simulink model "talos_navigation"  (R2023a)
settings: Solver=FixedStepDiscrete  StartTime=0.0  StopTime=10.0  FixedStep=1/1000.0  RelTol=1e-3  EnableMultiTasking=on
undefined symbols (not defined in the file): accel, child_frame_id, child_frame_id_SL_Info, data, data_SL_Info, header, layout, transform, transforms, transforms_SL_Info
libraries: ros2lib x187, simulink x9, sharedTrackingLibrary x1
(part 1 of 3)
settings Model: Creator=ethan  LastModifiedBy=ethan
settings OptimizationCC: DefaultParameterBehavior=Inlined  EnhancedBackFolding=on  PassReuseOutputArgsAs=Individual arguments  ZeroExternalMemoryAtStartup=off  ZeroInternalMemoryAtStartup=off  OptimizeBlockOrder=speed  DifferentSizesBufferReuse=on  OptimizationCustomize=off  EfficientTunableParamExpr=on
settings DebuggingCC: ParameterTunabilityLossMsg=error
settings SFSimCC: MATLABDynamicMemAlloc=off
settings RTWCC: Description=Embedded Coder  SystemTargetFile=ert.tlc  TemplateMakefile=ert_default_tmf  CustomInitializer=talos_nav_start_wake_timer();  CustomTerminator=talos_nav_release_ros();
settings RTWCC: CustomSourceCode=|
  | #include <chrono>
  | #include <new>
  | 
  | template<class T>
  | static void talos_nav_release(T & entity)
  | {
  |   entity.~T();
  |   new (&entity) T();
  | }
  | 
  | static rclcpp::CallbackGroup::SharedPtr talos_nav_wake_group;
  | static rclcpp::TimerBase::SharedPtr talos_nav_wake_timer;
  | 
  | static void talos_nav_start_wake_timer()
  | {
  |   talos_nav_wake_group = SLROSNodePtr->create_callback_group(rclcpp::CallbackGroupType::Reentrant);
  |   talos_nav_wake_timer = SLROSNodePtr->create_wall_timer(
  |     std::chrono::milliseconds(10), []() {}, talos_nav_wake_group);
  | }
  | 
  | static void talos_nav_release_ros()
  | {
  |   talos_nav_wake_timer.reset();
  |   talos_nav_wake_group.reset();
  |   talos_nav_release(Pub_talos_navigation_776);
  |   talos_nav_release(Pub_talos_navigation_825);
  |   talos_nav_release(Pub_talos_navigation_838);
  |   talos_nav_release(Pub_talos_navigation_751);
  |   talos_nav_release(Pub_talos_navigation_804);
  |   talos_nav_release(Sub_talos_navigation_275);
  |   talos_nav_release(Sub_talos_navigation_273);
  |   talos_nav_release(Sub_talos_navigation_271);
  |   talos_nav_release(Sub_talos_navigation_269);
  |   talos_nav_release(Sub_talos_navigation_277);
  |   talos_nav_release(ParamGet_talos_navigation_254);
  |   talos_nav_release(ParamGet_talos_navigation_252);
  |   talos_nav_release(ParamGet_talos_navigation_253);
  |   talos_nav_release(ParamGet_talos_navigation_255);
  |   talos_nav_release(ParamGet_talos_navigation_168);
  |   talos_nav_release(ParamGet_talos_navigation_171);
  |   talos_nav_release(ParamGet_talos_navigation_172);
  |   talos_nav_release(ParamGet_talos_navigation_173);
  |   talos_nav_release(ParamGet_talos_navigation_175);
  |   talos_nav_release(ParamGet_talos_navigation_177);
  |   talos_nav_release(ParamGet_talos_navigation_176);
  |   talos_nav_release(ParamGet_talos_navigation_167);
  |   talos_nav_release(ParamGet_talos_navigation_179);
  |   talos_nav_release(ParamGet_talos_navigation_178);
  |   talos_nav_release(ParamGet_talos_navigation_221);
  |   talos_nav_release(ParamGet_talos_navigation_219);
  |   talos_nav_release(ParamGet_talos_navigation_220);
  |   talos_nav_release(ParamGet_talos_navigation_218);
  |   talos_nav_release(ParamGet_talos_navigation_165);
  |   talos_nav_release(ParamGet_talos_navigation_182);
  |   talos_nav_release(ParamGet_talos_navigation_183);
  |   talos_nav_release(ParamGet_talos_navigation_192);
  |   talos_nav_release(ParamGet_talos_navigation_193);
  |   talos_nav_release(ParamGet_talos_navigation_194);
  |   talos_nav_release(ParamGet_talos_navigation_195);
  |   talos_nav_release(ParamGet_talos_navigation_196);
  |   talos_nav_release(ParamGet_talos_navigation_197);
  |   talos_nav_release(ParamGet_talos_navigation_184);
  |   talos_nav_release(ParamGet_talos_navigation_185);
  |   talos_nav_release(ParamGet_talos_navigation_186);
  |   talos_nav_release(ParamGet_talos_navigation_187);
  |   talos_nav_release(ParamGet_talos_navigation_188);
  |   talos_nav_release(ParamGet_talos_navigation_189);
  |   talos_nav_release(ParamGet_talos_navigation_190);
  |   talos_nav_release(ParamGet_talos_navigation_191);
  |   talos_nav_release(ParamGet_talos_navigation_201);
  |   talos_nav_release(ParamGet_talos_navigation_202);
  |   talos_nav_release(ParamGet_talos_navigation_211);
  |   talos_nav_release(ParamGet_talos_navigation_212);
  |   talos_nav_release(ParamGet_talos_navigation_213);
  |   talos_nav_release(ParamGet_talos_navigation_214);
  |   talos_nav_release(ParamGet_talos_navigation_215);
  |   talos_nav_release(ParamGet_talos_navigation_216);
  |   talos_nav_release(ParamGet_talos_navigation_203);
  |   talos_nav_release(ParamGet_talos_navigation_204);
  |   talos_nav_release(ParamGet_talos_navigation_205);
  |   talos_nav_release(ParamGet_talos_navigation_206);
  |   talos_nav_release(ParamGet_talos_navigation_207);
  |   talos_nav_release(ParamGet_talos_navigation_208);
  |   talos_nav_release(ParamGet_talos_navigation_209);
  |   talos_nav_release(ParamGet_talos_navigation_210);
  |   talos_nav_release(ParamGet_talos_navigation_222);
  |   talos_nav_release(ParamGet_talos_navigation_166);
  |   talos_nav_release(ParamGet_talos_navigation_7);
  |   talos_nav_release(ParamGet_talos_navigation_14);
  |   talos_nav_release(ParamGet_talos_navigation_12);
  |   talos_nav_release(ParamGet_talos_navigation_10);
  |   talos_nav_release(ParamGet_talos_navigation_9);
  |   talos_nav_release(ParamGet_talos_navigation_5);
  |   talos_nav_release(ParamGet_talos_navigation_227);
  |   talos_nav_release(ParamGet_talos_navigation_240);
  |   talos_nav_release(ParamGet_talos_navigation_226);
  |   talos_nav_release(ParamGet_talos_navigation_241);
  |   talos_nav_release(ParamGet_talos_navigation_242);
  |   talos_nav_release(ParamGet_talos_navigation_229);
  |   talos_nav_release(ParamGet_talos_navigation_230);
  |   talos_nav_release(ParamGet_talos_navigation_235);
  |   talos_nav_release(ParamGet_talos_navigation_236);
  |   talos_nav_release(ParamGet_talos_navigation_237);
  |   talos_nav_release(ParamGet_talos_navigation_238);
  |   talos_nav_release(ParamGet_talos_navigation_244);
  |   talos_nav_release(ParamGet_talos_navigation_248);
  |   talos_nav_release(ParamGet_talos_navigation_247);
  |   talos_nav_release(ParamGet_talos_navigation_243);
  |   talos_nav_release(ParamGet_talos_navigation_245);
  |   talos_nav_release(ParamGet_talos_navigation_246);
  |   talos_nav_release(ParamGet_talos_navigation_232);
  |   talos_nav_release(ParamGet_talos_navigation_228);
  |   talos_nav_release(ParamGet_talos_navigation_231);
  |   talos_nav_release(ParamGet_talos_navigation_62);
  |   talos_nav_release(ParamGet_talos_navigation_64);
  |   talos_nav_release(ParamGet_talos_navigation_73);
  |   talos_nav_release(ParamGet_talos_navigation_74);
  |   talos_nav_release(ParamGet_talos_navigation_75);
  |   talos_nav_release(ParamGet_talos_navigation_76);
  |   talos_nav_release(ParamGet_talos_navigation_67);
  |   talos_nav_release(ParamGet_talos_navigation_68);
  |   talos_nav_release(ParamGet_talos_navigation_69);
  |   talos_nav_release(ParamGet_talos_navigation_48);
  |   talos_nav_release(ParamGet_talos_navigation_57);
  |   talos_nav_release(ParamGet_talos_navigation_58);
  |   talos_nav_release(ParamGet_talos_navigation_59);
  |   talos_nav_release(ParamGet_talos_navigation_60);
  |   talos_nav_release(ParamGet_talos_navigation_51);
  |   talos_nav_release(ParamGet_talos_navigation_52);
  |   talos_nav_release(ParamGet_talos_navigation_53);
  |   talos_nav_release(ParamGet_talos_navigation_34);
  |   talos_nav_release(ParamGet_talos_navigation_43);
  |   talos_nav_release(ParamGet_talos_navigation_44);
  |   talos_nav_release(ParamGet_talos_navigation_45);
  |   talos_nav_release(ParamGet_talos_navigation_46);
  |   talos_nav_release(ParamGet_talos_navigation_37);
  |   talos_nav_release(ParamGet_talos_navigation_38);
  |   talos_nav_release(ParamGet_talos_navigation_39);
  |   talos_nav_release(ParamGet_talos_navigation_20);
  |   talos_nav_release(ParamGet_talos_navigation_29);
  |   talos_nav_release(ParamGet_talos_navigation_30);
  |   talos_nav_release(ParamGet_talos_navigation_31);
  |   talos_nav_release(ParamGet_talos_navigation_32);
  |   talos_nav_release(ParamGet_talos_navigation_23);
  |   talos_nav_release(ParamGet_talos_navigation_24);
  |   talos_nav_release(ParamGet_talos_navigation_25);
  |   talos_nav_release(ParamGet_talos_navigation_19);
  |   talos_nav_release(ParamGet_talos_navigation_153);
  |   talos_nav_release(ParamGet_talos_navigation_156);
  |   talos_nav_release(ParamGet_talos_navigation_155);
  |   talos_nav_release(ParamGet_talos_navigation_159);
  |   talos_nav_release(ParamGet_talos_navigation_158);
  |   talos_nav_release(ParamGet_talos_navigation_157);
  |   talos_nav_release(ParamGet_talos_navigation_154);
  |   talos_nav_release(ParamGet_talos_navigation_152);
  |   talos_nav_release(ParamGet_talos_navigation_114);
  |   talos_nav_release(ParamGet_talos_navigation_136);
  |   talos_nav_release(ParamGet_talos_navigation_137);
  |   talos_nav_release(ParamGet_talos_navigation_138);
  |   talos_nav_release(ParamGet_talos_navigation_151);
  |   talos_nav_release(ParamGet_talos_navigation_110);
  |   talos_nav_release(ParamGet_talos_navigation_142);
  |   talos_nav_release(ParamGet_talos_navigation_143);
  |   talos_nav_release(ParamGet_talos_navigation_144);
  |   talos_nav_release(ParamGet_talos_navigation_150);
  |   talos_nav_release(ParamGet_talos_navigation_112);
  |   talos_nav_release(ParamGet_talos_navigation_161);
  |   talos_nav_release(ParamGet_talos_navigation_130);
  |   talos_nav_release(ParamGet_talos_navigation_131);
  |   talos_nav_release(ParamGet_talos_navigation_132);
  |   talos_nav_release(ParamGet_talos_navigation_149);
  |   talos_nav_release(ParamGet_talos_navigation_124);
  |   talos_nav_release(ParamGet_talos_navigation_125);
  |   talos_nav_release(ParamGet_talos_navigation_126);
  |   talos_nav_release(ParamGet_talos_navigation_146);
  |   talos_nav_release(ParamGet_talos_navigation_118);
  |   talos_nav_release(ParamGet_talos_navigation_119);
  |   talos_nav_release(ParamGet_talos_navigation_120);
  |   talos_nav_release(ParamGet_talos_navigation_160);
  |   talos_nav_release(ParamGet_talos_navigation_147);
  |   talos_nav_release(ParamGet_talos_navigation_148);
  |   talos_nav_release(ParamGet_talos_navigation_108);
  |   talos_nav_release(ParamGet_talos_navigation_90);
  |   talos_nav_release(ParamGet_talos_navigation_81);
  |   talos_nav_release(ParamGet_talos_navigation_87);
  |   talos_nav_release(ParamGet_talos_navigation_88);
  |   talos_nav_release(ParamGet_talos_navigation_84);
  |   talos_nav_release(ParamGet_talos_navigation_100);
  |   talos_nav_release(ParamGet_talos_navigation_89);
  |   talos_nav_release(ParamGet_talos_navigation_85);
  |   talos_nav_release(ParamGet_talos_navigation_83);
  |   talos_nav_release(ParamGet_talos_navigation_86);
  |   talos_nav_release(ParamGet_talos_navigation_103);
  |   talos_nav_release(ParamGet_talos_navigation_101);
  |   talos_nav_release(ParamGet_talos_navigation_102);
  |   talos_nav_release(ParamGet_talos_navigation_104);
  |   talos_nav_release(ParamGet_talos_navigation_98);
  |   talos_nav_release(ParamGet_talos_navigation_82);
  |   talos_nav_release(ParamGet_talos_navigation_99);
  |   talos_nav_release(ParamGet_talos_navigation_93);
  |   talos_nav_release(ParamGet_talos_navigation_94);
  |   talos_nav_release(ParamGet_talos_navigation_95);
  |   talos_nav_release(ParamGet_talos_navigation_96);
  | }
settings RTWCC: CustomHeaderCode=|
  | #undef rtmStepTask
  | #define rtmStepTask(rtm, idx) ((idx) < 3 && (rtm)->Timing.TaskCounters.TID[(idx)] == 0)
  | #define step3 step2
settings CodeAppCC: ForceParamTrailComments=on  IgnoreCustomStorageClasses=off  OperatorAnnotations=on  SimulinkDataObjDesc=on  SFDataObjDesc=on  InsertBlockDesc=on
settings ERTTargetCC: TargetLangStandard=C99 (ISO)  GenerateSampleERTMain=on  SupportVariableSizeSignals=on  InlinedParameterPlacement=NonHierarchical  ERTCustomFileTemplate=example_file_process.tlc

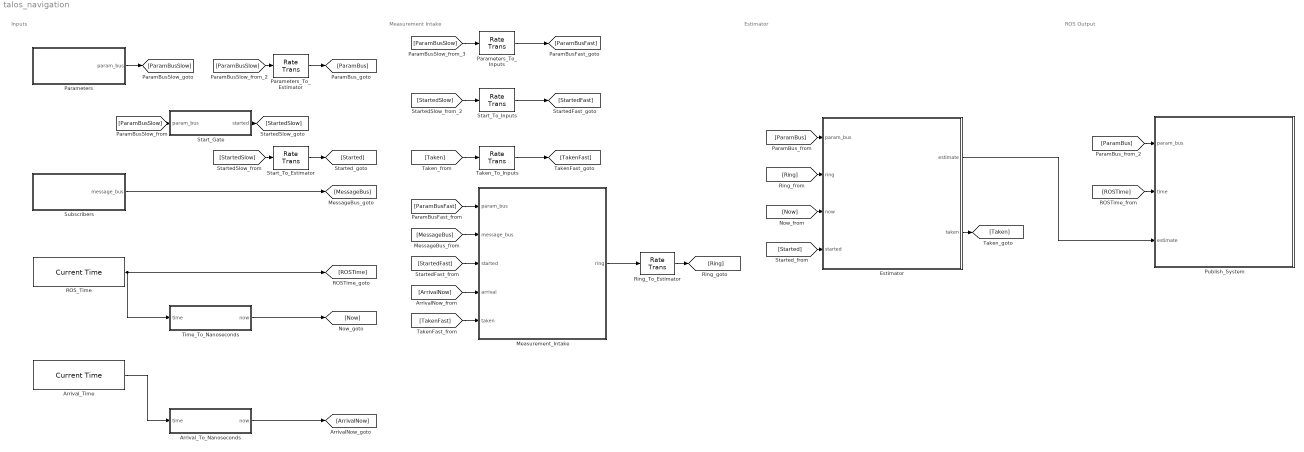
== system talos_navigation ==
  note: Inputs
  note: Measurement Intake
  note: Estimator
  note: ROS Output
  Arrival_Time : ros2lib/Current Time  OutputFormat=bus  SampleTime=1/1000.0  ModelName=untitled
  Arrival_To_Nanoseconds : Subsystem
  Estimator : Subsystem
  Measurement_Intake : Subsystem
  Parameters : Subsystem
  Parameters_To_Estimator : RateTransition  OutPortSampleTime=1/500.0
  Parameters_To_Inputs : RateTransition  OutPortSampleTime=1/1000.0
  Publish_System : Subsystem
  ROS_Time : ros2lib/Current Time  OutputFormat=bus  SampleTime=1/500.0  ModelName=untitled
  Ring_To_Estimator : RateTransition  Deterministic=off  OutPortSampleTime=1/500.0
  Start_Gate : Subsystem
  Start_To_Estimator : RateTransition  Deterministic=off  OutPortSampleTime=1/500.0
  Start_To_Inputs : RateTransition  Deterministic=off  OutPortSampleTime=1/1000.0
  Subscribers : Subsystem
  Taken_To_Inputs : RateTransition  Deterministic=off  OutPortSampleTime=1/1000.0
  Time_To_Nanoseconds : Subsystem
  wires:
  Parameters/1(param_bus) -> [ParamBusSlow]
  [ParamBusSlow] -> Start_Gate/1(param_bus)
  Start_Gate/1(started) -> [StartedSlow]
  [ParamBusSlow] -> Parameters_To_Estimator/1
  Parameters_To_Estimator/1 -> [ParamBus]
  [StartedSlow] -> Start_To_Estimator/1
  Start_To_Estimator/1 -> [Started]
  Subscribers/1(message_bus) -> [MessageBus]
  ROS_Time/1 -> [ROSTime], Time_To_Nanoseconds/1(time)
  Time_To_Nanoseconds/1(now) -> [Now]
  Arrival_Time/1 -> Arrival_To_Nanoseconds/1(time)
  Arrival_To_Nanoseconds/1(now) -> [ArrivalNow]
  [ParamBusSlow] -> Parameters_To_Inputs/1
  Parameters_To_Inputs/1 -> [ParamBusFast]
  [StartedSlow] -> Start_To_Inputs/1
  Start_To_Inputs/1 -> [StartedFast]
  [ParamBusFast] -> Measurement_Intake/1(param_bus)
  [MessageBus] -> Measurement_Intake/2(message_bus)
  [StartedFast] -> Measurement_Intake/3(started)
  [ArrivalNow] -> Measurement_Intake/4(arrival)
  [TakenFast] -> Measurement_Intake/5(taken)
  [Taken] -> Taken_To_Inputs/1
  Taken_To_Inputs/1 -> [TakenFast]
  Measurement_Intake/1(ring) -> Ring_To_Estimator/1
  Ring_To_Estimator/1 -> [Ring]
  [ParamBus] -> Estimator/1(param_bus)
  [Ring] -> Estimator/2(ring)
  [Now] -> Estimator/3(now)
  [Started] -> Estimator/4(started)
  Estimator/2(taken) -> [Taken]
  [ParamBus] -> Publish_System/1(param_bus)
  [ROSTime] -> Publish_System/2(time)
  Estimator/1(estimate) -> Publish_System/3(estimate)

== system talos_navigation/Arrival_To_Nanoseconds ==
  time : Inport
  nanosec_int64 : DataTypeConversion  OutDataTypeStr=int64  SaturateOnIntegerOverflow=off  RndMeth=Floor
  parts : BusSelector  OutputSignals=sec,nanosec
  per_second : Gain  Gain=1000000000  ParamDataTypeStr=int64  OutDataTypeStr=int64
  sec_int64 : DataTypeConversion  OutDataTypeStr=int64  SaturateOnIntegerOverflow=off  RndMeth=Floor
  total : Sum  OutDataTypeStr=int64
  now : Outport
  wires:
  time/1 -> parts/1
  parts/1 -> sec_int64/1  "<sec>"
  parts/2 -> nanosec_int64/1  "<nanosec>"
  sec_int64/1 -> per_second/1
  per_second/1 -> total/1
  nanosec_int64/1 -> total/2
  total/1 -> now/1  "now"

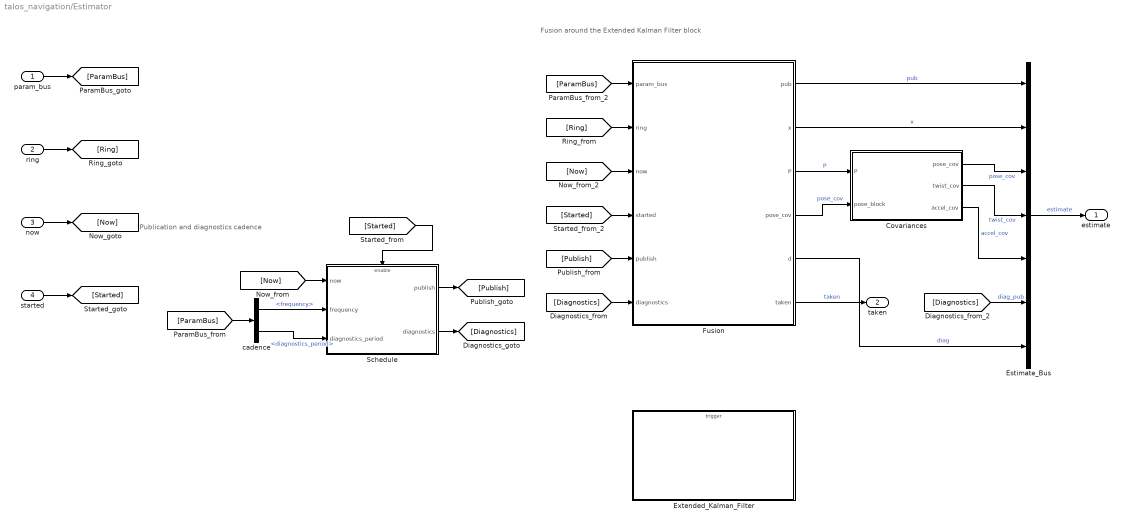
== system talos_navigation/Estimator ==
  note: Publication and diagnostics cadence
  note: Fusion around the Extended Kalman Filter block
  param_bus : Inport
  ring : Inport  Port=2
  now : Inport  Port=3
  started : Inport  Port=4
  Covariances : Subsystem
  Estimate_Bus : BusCreator  Inputs=7
  Extended_Kalman_Filter : Subsystem  TreatAsAtomicUnit=on
  Fusion : MATLAB Function  TreatAsAtomicUnit=on
  Schedule : Subsystem
  cadence : BusSelector  OutputSignals=timing.frequency,diagnostics.diagnostics_period
  estimate : Outport
  taken : Outport  Port=2
  wires:
  param_bus/1 -> [ParamBus]
  ring/1 -> [Ring]
  now/1 -> [Now]
  started/1 -> [Started]
  [Now] -> Schedule/1(now)
  [ParamBus] -> cadence/1
  [Started] -> Schedule/Enable
  cadence/1 -> Schedule/2(frequency)  "<frequency>"
  cadence/2 -> Schedule/3(diagnostics_period)  "<diagnostics_period>"
  Schedule/1(publish) -> [Publish]
  Schedule/2(diagnostics) -> [Diagnostics]
  [ParamBus] -> Fusion/1(param_bus)
  [Ring] -> Fusion/2(ring)
  [Now] -> Fusion/3(now)
  [Started] -> Fusion/4(started)
  [Publish] -> Fusion/5(publish)
  [Diagnostics] -> Fusion/6(diagnostics)
  Fusion/1(pub) -> Estimate_Bus/1  "pub"
  Fusion/2(x) -> Estimate_Bus/2  "x"
  Fusion/3(P) -> Covariances/1(P)  "P"
  Fusion/4(pose_cov) -> Covariances/2(pose_block)  "pose_cov"
  Covariances/1(pose_cov) -> Estimate_Bus/3  "pose_cov"
  Covariances/2(twist_cov) -> Estimate_Bus/4  "twist_cov"
  Covariances/3(accel_cov) -> Estimate_Bus/5  "accel_cov"
  [Diagnostics] -> Estimate_Bus/6  "diag_pub"
  Fusion/5(d) -> Estimate_Bus/7  "diag"
  Estimate_Bus/1 -> estimate/1  "estimate"
  Fusion/6(taken) -> taken/1  "taken"

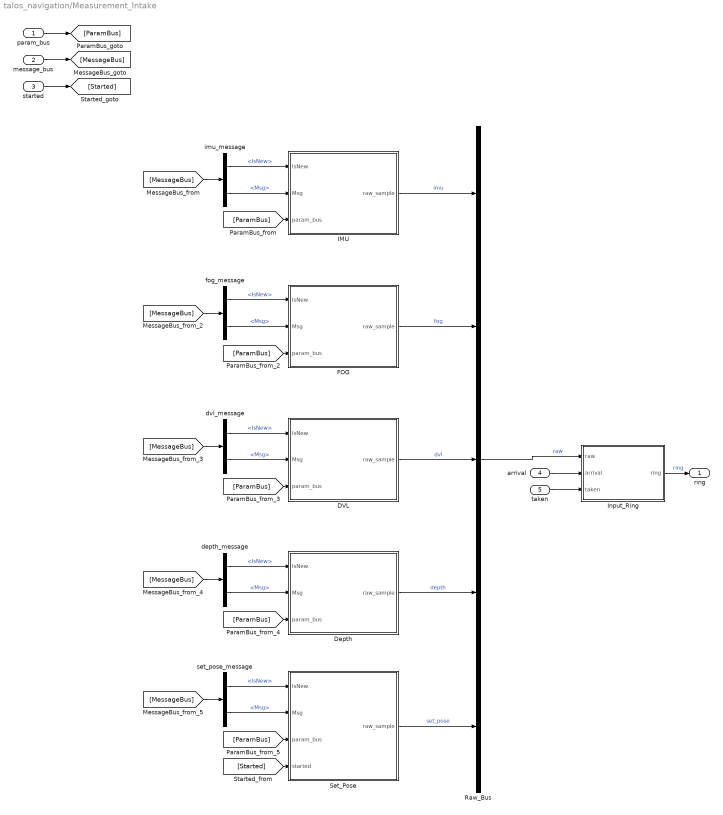
== system talos_navigation/Measurement_Intake ==
  param_bus : Inport
  message_bus : Inport  Port=2
  started : Inport  Port=3
  arrival : Inport  Port=4
  taken : Inport  Port=5
  DVL : Subsystem
  Depth : Subsystem
  FOG : Subsystem
  IMU : Subsystem
  Input_Ring : MATLAB Function  TreatAsAtomicUnit=on
  Raw_Bus : BusCreator  Inputs=5  OutDataTypeStr=Bus: talos_nav_raw  NonVirtualBus=on
  Set_Pose : Subsystem
  depth_message : BusSelector  OutputSignals=depth.IsNew,depth.Msg
  dvl_message : BusSelector  OutputSignals=dvl.IsNew,dvl.Msg
  fog_message : BusSelector  OutputSignals=fog.IsNew,fog.Msg
  imu_message : BusSelector  OutputSignals=imu.IsNew,imu.Msg
  set_pose_message : BusSelector  OutputSignals=set_pose.IsNew,set_pose.Msg
  ring : Outport
  wires:
  param_bus/1 -> [ParamBus]
  message_bus/1 -> [MessageBus]
  started/1 -> [Started]
  imu_message/1 -> IMU/1(IsNew)  "<IsNew>"
  imu_message/2 -> IMU/2(Msg)  "<Msg>"
  [MessageBus] -> imu_message/1
  [ParamBus] -> IMU/3(param_bus)
  IMU/1(raw_sample) -> Raw_Bus/1  "imu"
  fog_message/1 -> FOG/1(IsNew)  "<IsNew>"
  fog_message/2 -> FOG/2(Msg)  "<Msg>"
  [MessageBus] -> fog_message/1
  [ParamBus] -> FOG/3(param_bus)
  FOG/1(raw_sample) -> Raw_Bus/2  "fog"
  dvl_message/1 -> DVL/1(IsNew)  "<IsNew>"
  dvl_message/2 -> DVL/2(Msg)  "<Msg>"
  [MessageBus] -> dvl_message/1
  [ParamBus] -> DVL/3(param_bus)
  DVL/1(raw_sample) -> Raw_Bus/3  "dvl"
  depth_message/1 -> Depth/1(IsNew)  "<IsNew>"
  depth_message/2 -> Depth/2(Msg)  "<Msg>"
  [MessageBus] -> depth_message/1
  [ParamBus] -> Depth/3(param_bus)
  Depth/1(raw_sample) -> Raw_Bus/4  "depth"
  set_pose_message/1 -> Set_Pose/1(IsNew)  "<IsNew>"
  set_pose_message/2 -> Set_Pose/2(Msg)  "<Msg>"
  [MessageBus] -> set_pose_message/1
  [ParamBus] -> Set_Pose/3(param_bus)
  [Started] -> Set_Pose/4(started)
  Set_Pose/1(raw_sample) -> Raw_Bus/5  "set_pose"
  Raw_Bus/1 -> Input_Ring/1(raw)  "raw"
  arrival/1 -> Input_Ring/2(arrival)
  taken/1 -> Input_Ring/3(taken)
  Input_Ring/1(ring) -> ring/1  "ring"

== system talos_navigation/Parameters ==
  Param_Bus : BusCreator  Inputs=7  OutDataTypeStr=Bus: talos_nav_params  NonVirtualBus=on
  diagnostics : Subsystem
  estimator : Subsystem
  frames : Subsystem
  gates : Subsystem
  mounts : Subsystem
  sensor_axes : Subsystem
  timing : Subsystem
  param_bus : Outport
  wires:
  frames/1(frames) -> Param_Bus/1  "frames"
  mounts/1(mounts) -> Param_Bus/2  "mounts"
  timing/1(timing) -> Param_Bus/3  "timing"
  sensor_axes/1(sensor_axes) -> Param_Bus/4  "sensor_axes"
  estimator/1(estimator) -> Param_Bus/5  "estimator"
  gates/1(gates) -> Param_Bus/6  "gates"
  diagnostics/1(diagnostics) -> Param_Bus/7  "diagnostics"
  Param_Bus/1 -> param_bus/1

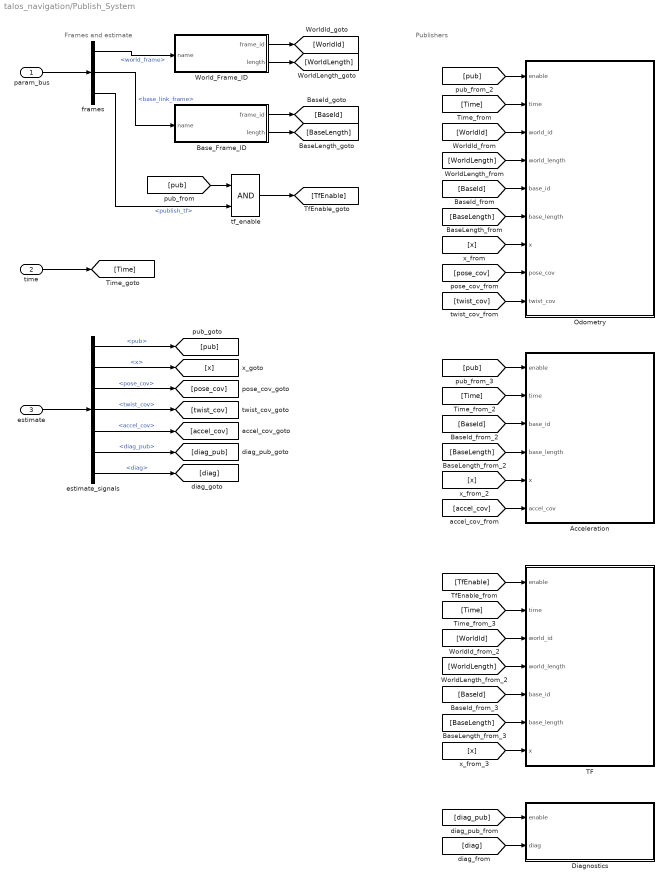
== system talos_navigation/Publish_System ==
  note: Frames and estimate
  note: Publishers
  param_bus : Inport
  time : Inport  Port=2
  estimate : Inport  Port=3
  Acceleration : Subsystem
  Base_Frame_ID : Subsystem
  Diagnostics : Subsystem
  Odometry : Subsystem
  TF : Subsystem
  World_Frame_ID : Subsystem
  estimate_signals : BusSelector  OutputSignals=pub,x,pose_cov,twist_cov,accel_cov,diag_pub,diag
  frames : BusSelector  OutputSignals=frames.world_frame,frames.base_link_frame,frames.publish_tf
  tf_enable : Logic  AllPortsSameDT=off  OutDataTypeStr=boolean
  wires:
  param_bus/1 -> frames/1
  estimate/1 -> estimate_signals/1
  frames/1 -> World_Frame_ID/1(name)  "<world_frame>"
  frames/2 -> Base_Frame_ID/1(name)  "<base_link_frame>"
  World_Frame_ID/1(frame_id) -> [WorldId]
  World_Frame_ID/2(length) -> [WorldLength]
  Base_Frame_ID/1(frame_id) -> [BaseId]
  Base_Frame_ID/2(length) -> [BaseLength]
  time/1 -> [Time]
  estimate_signals/1 -> [pub]  "<pub>"
  estimate_signals/2 -> [x]  "<x>"
  estimate_signals/3 -> [pose_cov]  "<pose_cov>"
  estimate_signals/4 -> [twist_cov]  "<twist_cov>"
  estimate_signals/5 -> [accel_cov]  "<accel_cov>"
  estimate_signals/6 -> [diag_pub]  "<diag_pub>"
  estimate_signals/7 -> [diag]  "<diag>"
  [pub] -> tf_enable/1
  frames/3 -> tf_enable/2  "<publish_tf>"
  tf_enable/1 -> [TfEnable]
  [pub] -> Odometry/1(enable)
  [Time] -> Odometry/2(time)
  [WorldId] -> Odometry/3(world_id)
  [WorldLength] -> Odometry/4(world_length)
  [BaseId] -> Odometry/5(base_id)
  [BaseLength] -> Odometry/6(base_length)
  [x] -> Odometry/7(x)
  [pose_cov] -> Odometry/8(pose_cov)
  [twist_cov] -> Odometry/9(twist_cov)
  [pub] -> Acceleration/1(enable)
  [Time] -> Acceleration/2(time)
  [BaseId] -> Acceleration/3(base_id)
  [BaseLength] -> Acceleration/4(base_length)
  [x] -> Acceleration/5(x)
  [accel_cov] -> Acceleration/6(accel_cov)
  [TfEnable] -> TF/1(enable)
  [Time] -> TF/2(time)
  [WorldId] -> TF/3(world_id)
  [WorldLength] -> TF/4(world_length)
  [BaseId] -> TF/5(base_id)
  [BaseLength] -> TF/6(base_length)
  [x] -> TF/7(x)
  [diag_pub] -> Diagnostics/1(enable)
  [diag] -> Diagnostics/2(diag)

== system talos_navigation/Start_Gate ==
  param_bus : Inport
  latch : Logic  Operator=OR  AllPortsSameDT=off  OutDataTypeStr=boolean
  loaded : BusSelector  OutputSignals=mounts.parameters_loaded
  loaded_before : UnitDelay  InitialCondition=false  SampleTime=-1  HasFrameUpgradeWarning=on
  started_before : UnitDelay  InitialCondition=false  SampleTime=-1  HasFrameUpgradeWarning=on
  twice : Logic  AllPortsSameDT=off  OutDataTypeStr=boolean
  started : Outport
  wires:
  param_bus/1 -> loaded/1
  loaded/1 -> twice/1, loaded_before/1  "<parameters_loaded>"
  loaded_before/1 -> twice/2
  twice/1 -> latch/1
  latch/1 -> started/1, started_before/1  "started"
  started_before/1 -> latch/2

== system talos_navigation/Subscribers ==
  Message_Bus : BusCreator  Inputs=5
  depth_bus : BusCreator  Inputs=2
  dvl_bus : BusCreator  Inputs=2
  fog_bus : BusCreator  Inputs=2
  imu_bus : BusCreator  Inputs=2
  set_pose_bus : BusCreator  Inputs=2
  sub_depth : ros2lib/Subscribe  topicSource=Select from ROS network  topic=depth/pose  messageType=geometry_msgs/PoseWithCovarianceStamped  sampleTime=1/1000.0  QOSHistory=Keep last  QOSDepth=100  QOSReliability=Best effort  QOSDurability=Volatile
  sub_dvl : ros2lib/Subscribe  topicSource=Select from ROS network  topic=dvl_twist  messageType=geometry_msgs/TwistWithCovarianceStamped  sampleTime=1/1000.0  QOSHistory=Keep last  QOSDepth=100  QOSReliability=Best effort  QOSDurability=Volatile
  sub_fog : ros2lib/Subscribe  topicSource=Select from ROS network  topic=gyro/twist  messageType=geometry_msgs/TwistWithCovarianceStamped  sampleTime=1/1000.0  QOSHistory=Keep last  QOSDepth=100  QOSReliability=Best effort  QOSDurability=Volatile
  sub_imu : ros2lib/Subscribe  topicSource=Select from ROS network  topic=vectornav/imu  messageType=sensor_msgs/Imu  sampleTime=1/1000.0  QOSHistory=Keep last  QOSDepth=100  QOSReliability=Best effort  QOSDurability=Volatile
  sub_set_pose : ros2lib/Subscribe  topicSource=Select from ROS network  topic=set_pose  messageType=geometry_msgs/PoseWithCovarianceStamped  sampleTime=1/1000.0  QOSHistory=Keep last  QOSDepth=100  QOSReliability=Best effort  QOSDurability=Volatile
  message_bus : Outport
  wires:
  sub_imu/1 -> imu_bus/1  "IsNew"
  sub_imu/2 -> imu_bus/2  "Msg"
  imu_bus/1 -> Message_Bus/1  "imu"
  sub_fog/1 -> fog_bus/1  "IsNew"
  sub_fog/2 -> fog_bus/2  "Msg"
  fog_bus/1 -> Message_Bus/2  "fog"
  sub_dvl/1 -> dvl_bus/1  "IsNew"
  sub_dvl/2 -> dvl_bus/2  "Msg"
  dvl_bus/1 -> Message_Bus/3  "dvl"
  sub_depth/1 -> depth_bus/1  "IsNew"
  sub_depth/2 -> depth_bus/2  "Msg"
  depth_bus/1 -> Message_Bus/4  "depth"
  sub_set_pose/1 -> set_pose_bus/1  "IsNew"
  sub_set_pose/2 -> set_pose_bus/2  "Msg"
  set_pose_bus/1 -> Message_Bus/5  "set_pose"
  Message_Bus/1 -> message_bus/1

== system talos_navigation/Time_To_Nanoseconds ==
  time : Inport
  nanosec_int64 : DataTypeConversion  OutDataTypeStr=int64  SaturateOnIntegerOverflow=off  RndMeth=Floor
  parts : BusSelector  OutputSignals=sec,nanosec
  per_second : Gain  Gain=1000000000  ParamDataTypeStr=int64  OutDataTypeStr=int64
  sec_int64 : DataTypeConversion  OutDataTypeStr=int64  SaturateOnIntegerOverflow=off  RndMeth=Floor
  total : Sum  OutDataTypeStr=int64
  now : Outport
  wires:
  time/1 -> parts/1
  parts/1 -> sec_int64/1  "<sec>"
  parts/2 -> nanosec_int64/1  "<nanosec>"
  sec_int64/1 -> per_second/1
  per_second/1 -> total/1
  nanosec_int64/1 -> total/2
  total/1 -> now/1  "now"

== system talos_navigation/Estimator/Covariances ==
  P : Inport
  pose_block : Inport  Port=2
  accel_block : Selector  NumberOfDimensions=2  InputPortWidth=3  IndexOptions=Index vector (dialog),Index vector (dialog)  Indices=14:16,14:16  OutputSizes=1
  accel_row_major : Reshape
  accel_rows : Math  Operator=transpose
  pad_columns : Concatenate  Mode=Multidimensional array  ConcatenateDimension=2
  pad_rows : Concatenate  Mode=Multidimensional array
  pose_row_major : Reshape
  pose_rows : Math  Operator=transpose
  twist_block : Selector  NumberOfDimensions=2  InputPortWidth=3  IndexOptions=Index vector (dialog),Index vector (dialog)  Indices=8:13,8:13  OutputSizes=1
  twist_row_major : Reshape
  twist_rows : Math  Operator=transpose
  zeros_3x3 : Constant  Value=zeros(3)
  zeros_3x6 : Constant  Value=zeros(3, 6)
  pose_cov : Outport
  twist_cov : Outport  Port=2
  accel_cov : Outport  Port=3
  wires:
  P/1 -> twist_block/1, accel_block/1
  accel_block/1 -> pad_columns/1
  zeros_3x3/1 -> pad_columns/2
  pad_columns/1 -> pad_rows/1
  zeros_3x6/1 -> pad_rows/2
  pose_block/1 -> pose_rows/1
  pose_rows/1 -> pose_row_major/1
  pose_row_major/1 -> pose_cov/1  "pose_cov"
  twist_block/1 -> twist_rows/1
  twist_rows/1 -> twist_row_major/1
  twist_row_major/1 -> twist_cov/1  "twist_cov"
  pad_rows/1 -> accel_rows/1
  accel_rows/1 -> accel_row_major/1
  accel_row_major/1 -> accel_cov/1  "accel_cov"

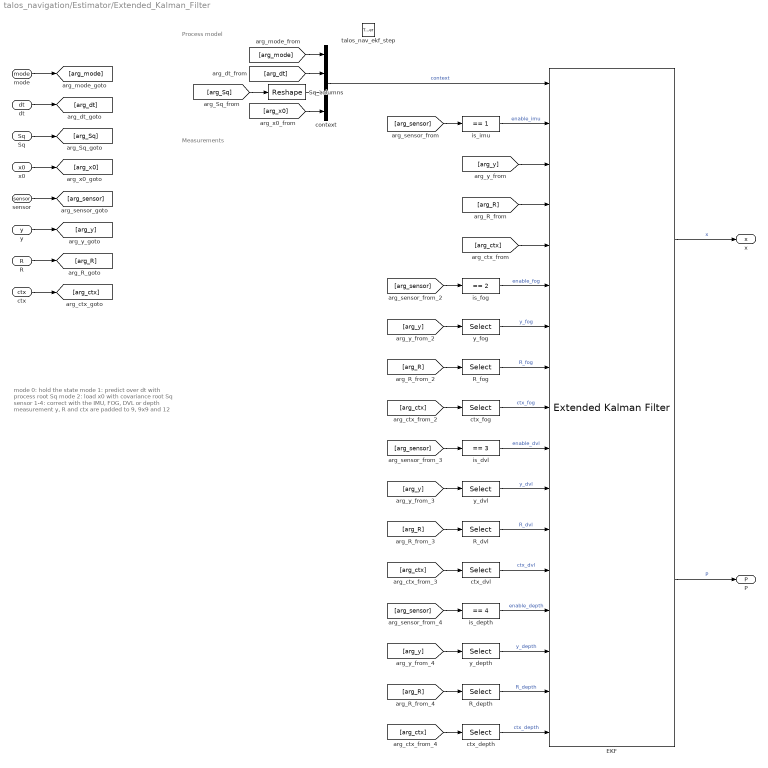
== system talos_navigation/Estimator/Extended_Kalman_Filter ==
  note: mode 0: hold the state
      | mode 1: predict over dt with process root Sq
      | mode 2: load x0 with covariance root Sq
      | sensor 1-4: correct with the IMU, FOG,
      | DVL or depth measurement
      | y, R and ctx are padded to 9, 9x9 and 12
  note: Process model
  note: Measurements
  talos_nav_ekf_step : TriggerPort  TriggerType=function-call  IsSimulinkFunction=on  FunctionName=talos_nav_ekf_step  FunctionVisibility=scoped  VariantControl=(inherit)
  EKF : sharedTrackingLibrary/Extended Kalman Filter  StateTransitionFcn=talos_nav_transition  HasStateTransitionJacobianFcn=on  StateTransitionJacobianFcn=talos_nav_transition_jacobian  HasAdditiveProcessNoise=Nonadditive  ProcessNoise=eye(19)  HasTimeVaryingProcessNoise=off  HasStateTransitionFcnExtraArgument=1  InitialState=[zeros(3, 1); 1; zeros(15, 1)]  InitialStateCovariance=eye(19)  MeasurementFcn1=talos_measure_imu_configured  HasMeasurementJacobianFcn1=on  MeasurementJacobianFcn1=talos_measure_imu_configured_jacobian  HasMeasurementEnablePort1=on  HasAdditiveMeasurementNoise1=Additive  MeasurementNoise1=1  HasTimeVaryingMeasurementNoise1=on  HasMeasurementFcnExtraArgument1=1  HasMeasurementWrapping1=off  MeasurementFcn2=talos_measure_fog_configured  HasMeasurementJacobianFcn2=on  MeasurementJacobianFcn2=talos_measure_fog_configured_jacobian  HasMeasurementEnablePort2=on  HasAdditiveMeasurementNoise2=Additive  MeasurementNoise2=1  HasTimeVaryingMeasurementNoise2=on  HasMeasurementFcnExtraArgument2=1  HasMeasurementWrapping2=off  MeasurementFcn3=talos_measure_dvl_configured  HasMeasurementJacobianFcn3=on  MeasurementJacobianFcn3=talos_measure_dvl_configured_jacobian  HasMeasurementEnablePort3=on  HasAdditiveMeasurementNoise3=Additive  MeasurementNoise3=1  HasTimeVaryingMeasurementNoise3=on  HasMeasurementFcnExtraArgument3=1  HasMeasurementWrapping3=off  MeasurementFcn4=talos_measure_depth_configured  HasMeasurementJacobianFcn4=on  MeasurementJacobianFcn4=talos_measure_depth_configured_jacobian  HasMeasurementEnablePort4=on  HasAdditiveMeasurementNoise4=Additive  MeasurementNoise4=1  HasTimeVaryingMeasurementNoise4=on  HasMeasurementFcnExtraArgument4=1  HasMeasurementWrapping4=off  HasMeasurementJacobianFcn5=off  HasMeasurementEnablePort5=off  HasAdditiveMeasurementNoise5=Additive  MeasurementNoise5=1  HasTimeVaryingMeasurementNoise5=off  HasMeasurementFcnExtraArgument5=0  HasMeasurementWrapping5=off  EnableMultirate=off  StateTransitionFcnSampleTime=1  MeasurementFcn1SampleTime=1  MeasurementFcn2SampleTime=1  MeasurementFcn3SampleTime=1  MeasurementFcn4SampleTime=1  MeasurementFcn5SampleTime=1  UseCurrentEstimator=on  OutputStateCovariance=on  DataType=double  SampleTime=-1  NumberOfMeasurements=4
  R_depth : Selector  NumberOfDimensions=2  InputPortWidth=3  IndexOptions=Index vector (dialog),Index vector (dialog)  Indices=1:1,1:1  OutputSizes=1
  R_dvl : Selector  NumberOfDimensions=2  InputPortWidth=3  IndexOptions=Index vector (dialog),Index vector (dialog)  Indices=1:3,1:3  OutputSizes=1
  R_fog : Selector  NumberOfDimensions=2  InputPortWidth=3  IndexOptions=Index vector (dialog),Index vector (dialog)  Indices=1:3,1:3  OutputSizes=1
  Sq_columns : Reshape
  context : Concatenate  NumInputs=4
  ctx_depth : Selector  InputPortWidth=12  IndexOptions=Index vector (dialog)  Indices=1:1  OutputSizes=1
  ctx_dvl : Selector  InputPortWidth=12  IndexOptions=Index vector (dialog)  Indices=1:6  OutputSizes=1
  ctx_fog : Selector  InputPortWidth=12  IndexOptions=Index vector (dialog)  Indices=1:3  OutputSizes=1
  is_depth : simulink/Logic and Bit Operations/Compare To Constant  relop===  const=4  OutDataTypeStr=boolean
  is_dvl : simulink/Logic and Bit Operations/Compare To Constant  relop===  const=3  OutDataTypeStr=boolean
  is_fog : simulink/Logic and Bit Operations/Compare To Constant  relop===  const=2  OutDataTypeStr=boolean
  is_imu : simulink/Logic and Bit Operations/Compare To Constant  relop===  const=1  OutDataTypeStr=boolean
  y_depth : Selector  InputPortWidth=9  IndexOptions=Index vector (dialog)  Indices=1:1  OutputSizes=1
  y_dvl : Selector  InputPortWidth=9  IndexOptions=Index vector (dialog)  Indices=1:3  OutputSizes=1
  y_fog : Selector  InputPortWidth=9  IndexOptions=Index vector (dialog)  Indices=1:3  OutputSizes=1
  mode : ArgIn  DisableCoverage=on  ArgumentName=mode
  dt : ArgIn  Port=2  ArgumentName=dt
  Sq : ArgIn  Port=3  PortDimensions=[19 19]  ArgumentName=Sq
  x0 : ArgIn  Port=4  PortDimensions=19  ArgumentName=x0
  sensor : ArgIn  Port=5  ArgumentName=sensor
  y : ArgIn  Port=6  PortDimensions=9  ArgumentName=y
  R : ArgIn  Port=7  PortDimensions=[9 9]  ArgumentName=R
  ctx : ArgIn  Port=8  PortDimensions=12  ArgumentName=ctx
  x : ArgOut  DisableCoverage=on  PortDimensions=19  ArgumentName=x
  P : ArgOut  Port=2  PortDimensions=[19 19]  ArgumentName=P
  wires:
  mode/1 -> [arg_mode]
  dt/1 -> [arg_dt]
  Sq/1 -> [arg_Sq]
  x0/1 -> [arg_x0]
  sensor/1 -> [arg_sensor]
  y/1 -> [arg_y]
  R/1 -> [arg_R]
  ctx/1 -> [arg_ctx]
  [arg_mode] -> context/1
  [arg_dt] -> context/2
  [arg_Sq] -> Sq_columns/1
  [arg_x0] -> context/4
  Sq_columns/1 -> context/3
  context/1 -> EKF/1  "context"
  [arg_sensor] -> is_imu/1
  is_imu/1 -> EKF/2  "enable_imu"
  [arg_y] -> EKF/3
  [arg_R] -> EKF/4
  [arg_ctx] -> EKF/5
  [arg_sensor] -> is_fog/1
  is_fog/1 -> EKF/6  "enable_fog"
  [arg_y] -> y_fog/1
  [arg_R] -> R_fog/1
  [arg_ctx] -> ctx_fog/1
  y_fog/1 -> EKF/7  "y_fog"
  R_fog/1 -> EKF/8  "R_fog"
  ctx_fog/1 -> EKF/9  "ctx_fog"
  [arg_sensor] -> is_dvl/1
  is_dvl/1 -> EKF/10  "enable_dvl"
  [arg_y] -> y_dvl/1
  [arg_R] -> R_dvl/1
  [arg_ctx] -> ctx_dvl/1
  y_dvl/1 -> EKF/11  "y_dvl"
  R_dvl/1 -> EKF/12  "R_dvl"
  ctx_dvl/1 -> EKF/13  "ctx_dvl"
  [arg_sensor] -> is_depth/1
  is_depth/1 -> EKF/14  "enable_depth"
  [arg_y] -> y_depth/1
  [arg_R] -> R_depth/1
  [arg_ctx] -> ctx_depth/1
  y_depth/1 -> EKF/15  "y_depth"
  R_depth/1 -> EKF/16  "R_depth"
  ctx_depth/1 -> EKF/17  "ctx_depth"
  EKF/1 -> x/1  "x"
  EKF/2 -> P/1  "P"

== system talos_navigation/Estimator/Schedule ==
  now : Inport
  frequency : Inport  Port=2
  diagnostics_period : Inport  Port=3
  started : EnablePort
  Diagnostics_Clock : Subsystem
  Publication_Clock : Subsystem
  publish : Outport  OutputWhenDisabled=reset  InitialOutput=false
  diagnostics : Outport  Port=2  OutputWhenDisabled=reset  InitialOutput=false
  wires:
  now/1 -> [Now]
  [Now] -> Publication_Clock/1(now)
  [Now] -> Diagnostics_Clock/1(now)
  frequency/1 -> Publication_Clock/2(frequency)
  diagnostics_period/1 -> Diagnostics_Clock/2(period_s)
  Publication_Clock/1(is_due) -> publish/1  "publish"
  Diagnostics_Clock/1(is_due) -> diagnostics/1  "diagnostics"

== system talos_navigation/Measurement_Intake/DVL ==
  IsNew : Inport
  Msg : Inport  Port=2
  param_bus : Inport  Port=3
  Frame_Kind : MATLAB Function  TreatAsAtomicUnit=on
  cov : Selector  NumberOfDimensions=2  InputPortWidth=3  IndexOptions=Index vector (dialog),Index vector (dialog)  Indices=1:3,1:3  OutputSizes=1
  cov_matrix : Reshape  OutputDimensionality=Customize  OutputDimensions=[6 6]
  cov_rows : Math  Operator=transpose
  fields : BusSelector  OutputSignals=header.stamp,twist.twist.linear.x,twist.twist.linear.y,twist.twist.linear.z,twist.covariance
  frame_fields : BusSelector  OutputSignals=header.frame_id,header.frame_id_SL_Info.CurrentLength
  frame_params : BusSelector  OutputSignals=frames.base_link_frame,frames.dvl_frame_fallback
  sample : BusCreator  Inputs=5  OutDataTypeStr=Bus: talos_nav_raw_dvl  NonVirtualBus=on
  stamp : Subsystem
  vel : Concatenate  NumInputs=3
  raw_sample : Outport
  wires:
  Msg/1 -> fields/1, frame_fields/1
  param_bus/1 -> frame_params/1
  fields/1 -> stamp/1(stamp)  "<stamp>"
  fields/2 -> vel/1  "<x>"
  fields/3 -> vel/2  "<y>"
  fields/4 -> vel/3  "<z>"
  fields/5 -> cov_matrix/1  "<covariance>"
  cov_matrix/1 -> cov_rows/1
  cov_rows/1 -> cov/1
  frame_fields/1 -> Frame_Kind/1(frame_id)  "<frame_id>"
  frame_fields/2 -> Frame_Kind/2(n)  "<CurrentLength>"
  frame_params/1 -> Frame_Kind/3(base)  "<base_link_frame>"
  frame_params/2 -> Frame_Kind/4(mount)  "<dvl_frame_fallback>"
  IsNew/1 -> sample/1  "valid"
  stamp/1(ns) -> sample/2  "stamp"
  vel/1 -> sample/3  "vel"
  cov/1 -> sample/4  "cov"
  Frame_Kind/1(frame) -> sample/5  "frame"
  sample/1 -> raw_sample/1

== system talos_navigation/Measurement_Intake/Depth ==
  IsNew : Inport
  Msg : Inport  Port=2
  param_bus : Inport  Port=3
  Depth_Mount : Subsystem
  Frame_Kind : MATLAB Function  TreatAsAtomicUnit=on
  fields : BusSelector  OutputSignals=header.stamp,pose.pose.position.x,pose.pose.position.y,pose.pose.position.z,pose.covariance
  frame_fields : BusSelector  OutputSignals=header.frame_id,header.frame_id_SL_Info.CurrentLength
  frame_params : BusSelector  OutputSignals=frames.base_link_frame,frames.world_frame,mounts.depth_frame,mounts.depth_mount_valid,mounts.depth_rotation,mounts.depth_translation
  position : Concatenate  NumInputs=3
  sample : BusCreator  Inputs=5  OutDataTypeStr=Bus: talos_nav_raw_depth  NonVirtualBus=on
  stamp : Subsystem
  variance : Selector  InputPortWidth=36  IndexOptions=Index vector (dialog)  Indices=15  OutputSizes=1
  raw_sample : Outport
  wires:
  Msg/1 -> fields/1, frame_fields/1
  param_bus/1 -> frame_params/1
  fields/1 -> stamp/1(stamp)  "<stamp>"
  fields/2 -> position/1  "<x>"
  fields/3 -> position/2  "<y>"
  fields/4 -> position/3  "<z>"
  fields/5 -> variance/1  "<covariance>"
  frame_fields/1 -> Frame_Kind/1(frame_id)  "<frame_id>"
  frame_fields/2 -> Frame_Kind/2(n)  "<CurrentLength>"
  frame_params/1 -> Frame_Kind/3(base)  "<base_link_frame>"
  frame_params/2 -> Frame_Kind/4(world)  "<world_frame>"
  frame_params/3 -> Frame_Kind/5(depth_frame)  "<depth_frame>"
  position/1 -> Depth_Mount/1(position)  "position"
  Frame_Kind/1(frame) -> Depth_Mount/2(kind)  "kind"
  Frame_Kind/2(mount) -> Depth_Mount/3(in_depth_frame)  "in_depth_frame"
  frame_params/4 -> Depth_Mount/4(mount_valid)  "<depth_mount_valid>"
  frame_params/5 -> Depth_Mount/5(rotation)  "<depth_rotation>"
  frame_params/6 -> Depth_Mount/6(translation)  "<depth_translation>"
  IsNew/1 -> sample/1  "valid"
  stamp/1(ns) -> sample/2  "stamp"
  Depth_Mount/1(z_world) -> sample/3  "z"
  variance/1 -> sample/4  "var"
  Depth_Mount/2(frame_world) -> sample/5  "frame"
  sample/1 -> raw_sample/1

== system talos_navigation/Measurement_Intake/FOG ==
  IsNew : Inport
  Msg : Inport  Port=2
  param_bus : Inport  Port=3
  Frame_Kind : MATLAB Function  TreatAsAtomicUnit=on
  cov : Selector  NumberOfDimensions=2  InputPortWidth=3  IndexOptions=Index vector (dialog),Index vector (dialog)  Indices=4:6,4:6  OutputSizes=1
  cov_matrix : Reshape  OutputDimensionality=Customize  OutputDimensions=[6 6]
  cov_rows : Math  Operator=transpose
  fields : BusSelector  OutputSignals=header.stamp,twist.twist.angular.x,twist.twist.angular.y,twist.twist.angular.z,twist.covariance
  frame_fields : BusSelector  OutputSignals=header.frame_id,header.frame_id_SL_Info.CurrentLength
  frame_params : BusSelector  OutputSignals=frames.base_link_frame,frames.fog_frame_fallback
  omega : Concatenate  NumInputs=3
  sample : BusCreator  Inputs=5  OutDataTypeStr=Bus: talos_nav_raw_fog  NonVirtualBus=on
  stamp : Subsystem
  raw_sample : Outport
  wires:
  Msg/1 -> fields/1, frame_fields/1
  param_bus/1 -> frame_params/1
  fields/1 -> stamp/1(stamp)  "<stamp>"
  fields/2 -> omega/1  "<x>"
  fields/3 -> omega/2  "<y>"
  fields/4 -> omega/3  "<z>"
  fields/5 -> cov_matrix/1  "<covariance>"
  cov_matrix/1 -> cov_rows/1
  cov_rows/1 -> cov/1
  frame_fields/1 -> Frame_Kind/1(frame_id)  "<frame_id>"
  frame_fields/2 -> Frame_Kind/2(n)  "<CurrentLength>"
  frame_params/1 -> Frame_Kind/3(base)  "<base_link_frame>"
  frame_params/2 -> Frame_Kind/4(mount)  "<fog_frame_fallback>"
  IsNew/1 -> sample/1  "valid"
  stamp/1(ns) -> sample/2  "stamp"
  omega/1 -> sample/3  "omega"
  cov/1 -> sample/4  "cov"
  Frame_Kind/1(frame) -> sample/5  "frame"
  sample/1 -> raw_sample/1

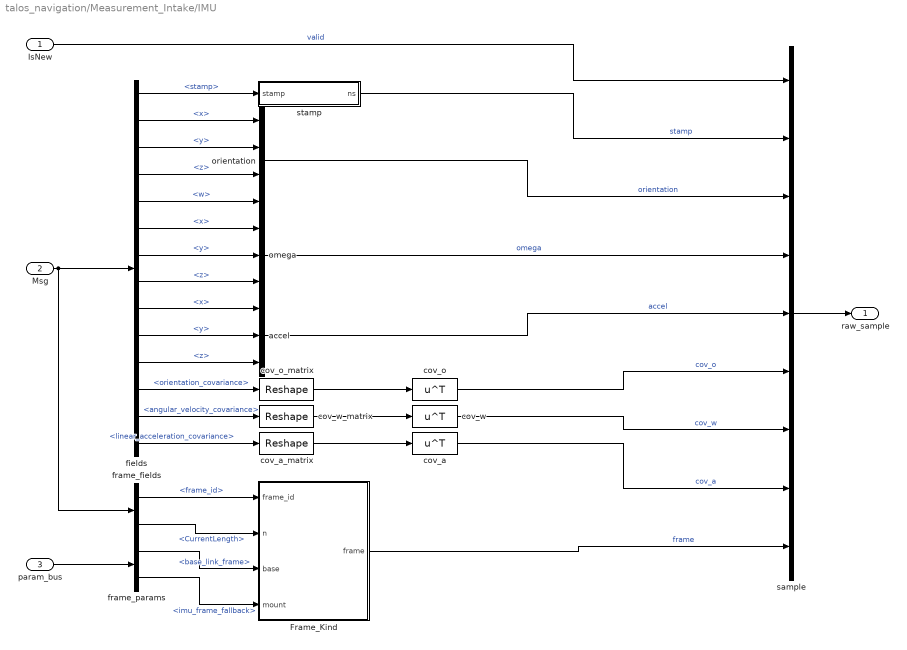
== system talos_navigation/Measurement_Intake/IMU ==
  IsNew : Inport
  Msg : Inport  Port=2
  param_bus : Inport  Port=3
  Frame_Kind : MATLAB Function  TreatAsAtomicUnit=on
  accel : Concatenate  NumInputs=3
  cov_a : Math  Operator=transpose
  cov_a_matrix : Reshape  OutputDimensionality=Customize  OutputDimensions=[3 3]
  cov_o : Math  Operator=transpose
  cov_o_matrix : Reshape  OutputDimensionality=Customize  OutputDimensions=[3 3]
  cov_w : Math  Operator=transpose
  cov_w_matrix : Reshape  OutputDimensionality=Customize  OutputDimensions=[3 3]
  fields : BusSelector  OutputSignals=header.stamp,orientation.x,orientation.y,orientation.z,orientation.w,angular_velocity.x,angular_velocity.y,angular_velocity.z,linear_acceleration.x,linear_acceleration.y,linear_acceleration.z,orientation_covariance,angular_velocity_covariance,linear_acceleration_covariance
  frame_fields : BusSelector  OutputSignals=header.frame_id,header.frame_id_SL_Info.CurrentLength
  frame_params : BusSelector  OutputSignals=frames.base_link_frame,frames.imu_frame_fallback
  omega : Concatenate  NumInputs=3
  orientation : Concatenate  NumInputs=4
  sample : BusCreator  Inputs=9  OutDataTypeStr=Bus: talos_nav_raw_imu  NonVirtualBus=on
  stamp : Subsystem
  raw_sample : Outport
  wires:
  Msg/1 -> fields/1, frame_fields/1
  param_bus/1 -> frame_params/1
  fields/1 -> stamp/1(stamp)  "<stamp>"
  fields/2 -> orientation/1  "<x>"
  fields/3 -> orientation/2  "<y>"
  fields/4 -> orientation/3  "<z>"
  fields/5 -> orientation/4  "<w>"
  fields/6 -> omega/1  "<x>"
  fields/7 -> omega/2  "<y>"
  fields/8 -> omega/3  "<z>"
  fields/9 -> accel/1  "<x>"
  fields/10 -> accel/2  "<y>"
  fields/11 -> accel/3  "<z>"
  fields/12 -> cov_o_matrix/1  "<orientation_covariance>"
  cov_o_matrix/1 -> cov_o/1
  fields/13 -> cov_w_matrix/1  "<angular_velocity_covariance>"
  cov_w_matrix/1 -> cov_w/1
  fields/14 -> cov_a_matrix/1  "<linear_acceleration_covariance>"
  cov_a_matrix/1 -> cov_a/1
  frame_fields/1 -> Frame_Kind/1(frame_id)  "<frame_id>"
  frame_fields/2 -> Frame_Kind/2(n)  "<CurrentLength>"
  frame_params/1 -> Frame_Kind/3(base)  "<base_link_frame>"
  frame_params/2 -> Frame_Kind/4(mount)  "<imu_frame_fallback>"
  IsNew/1 -> sample/1  "valid"
  stamp/1(ns) -> sample/2  "stamp"
  orientation/1 -> sample/3  "orientation"
  omega/1 -> sample/4  "omega"
  accel/1 -> sample/5  "accel"
  cov_o/1 -> sample/6  "cov_o"
  cov_w/1 -> sample/7  "cov_w"
  cov_a/1 -> sample/8  "cov_a"
  Frame_Kind/1(frame) -> sample/9  "frame"
  sample/1 -> raw_sample/1

== system talos_navigation/Measurement_Intake/Set_Pose ==
  IsNew : Inport
  Msg : Inport  Port=2
  param_bus : Inport  Port=3
  started : Inport  Port=4
  Frame_Kind : MATLAB Function  TreatAsAtomicUnit=on
  Hold_Until_Start : Subsystem
  cov : Math  Operator=transpose
  cov_matrix : Reshape  OutputDimensionality=Customize  OutputDimensions=[6 6]
  fields : BusSelector  OutputSignals=header.stamp,pose.pose.position.x,pose.pose.position.y,pose.pose.position.z,pose.pose.orientation.w,pose.pose.orientation.x,pose.pose.orientation.y,pose.pose.orientation.z,pose.covariance
  frame_fields : BusSelector  OutputSignals=header.frame_id,header.frame_id_SL_Info.CurrentLength
  frame_params : BusSelector  OutputSignals=frames.base_link_frame,frames.world_frame
  pos : Concatenate  NumInputs=3
  quat : Concatenate  NumInputs=4
  sample : BusCreator  Inputs=6  OutDataTypeStr=Bus: talos_nav_raw_set_pose  NonVirtualBus=on
  stamp : Subsystem
  raw_sample : Outport
  wires:
  IsNew/1 -> Hold_Until_Start/1(IsNew)
  Msg/1 -> Hold_Until_Start/2(Msg)
  started/1 -> Hold_Until_Start/3(started)
  Hold_Until_Start/2(msg) -> fields/1, frame_fields/1
  param_bus/1 -> frame_params/1
  fields/1 -> stamp/1(stamp)  "<stamp>"
  fields/2 -> pos/1  "<x>"
  fields/3 -> pos/2  "<y>"
  fields/4 -> pos/3  "<z>"
  fields/5 -> quat/1  "<w>"
  fields/6 -> quat/2  "<x>"
  fields/7 -> quat/3  "<y>"
  fields/8 -> quat/4  "<z>"
  fields/9 -> cov_matrix/1  "<covariance>"
  cov_matrix/1 -> cov/1
  frame_fields/1 -> Frame_Kind/1(frame_id)  "<frame_id>"
  frame_fields/2 -> Frame_Kind/2(n)  "<CurrentLength>"
  frame_params/1 -> Frame_Kind/3(base)  "<base_link_frame>"
  frame_params/2 -> Frame_Kind/4(world)  "<world_frame>"
  Hold_Until_Start/1(valid) -> sample/1  "valid"
  stamp/1(ns) -> sample/2  "stamp"
  pos/1 -> sample/3  "pos"
  quat/1 -> sample/4  "quat"
  cov/1 -> sample/5  "cov"
  Frame_Kind/1(frame) -> sample/6  "frame"
  sample/1 -> raw_sample/1

== system talos_navigation/Parameters/diagnostics ==
  diagnostics_bus : BusCreator  Inputs=4  OutDataTypeStr=Bus: talos_nav_params_diagnostics  NonVirtualBus=on
  diagnostics_period : ros2lib/Get Parameter  ParameterName=navigation__diagnostics__diagnostics_period  ParameterType=double  ParameterMaxArrayLength=16  ParameterInitialValue=1  SampleTime=1/10.0  ModelName=ros2lib  BlockId=ParamGet_ros2lib_196
  heading_std_warning : ros2lib/Get Parameter  ParameterName=navigation__diagnostics__heading_std_warning  ParameterType=double  ParameterMaxArrayLength=16  ParameterInitialValue=30  SampleTime=1/10.0  ModelName=ros2lib  BlockId=ParamGet_ros2lib_196
  position_offset_warning : ros2lib/Get Parameter  ParameterName=navigation__diagnostics__position_offset_warning  ParameterType=double  ParameterMaxArrayLength=16  ParameterInitialValue=0.05  SampleTime=1/10.0  ModelName=ros2lib  BlockId=ParamGet_ros2lib_196
  publish_debug_diagnostics : ros2lib/Get Parameter  ParameterName=navigation__diagnostics__publish_debug_diagnostics  ParameterType=boolean  ParameterMaxArrayLength=16  ParameterInitialValue=1  SampleTime=1/10.0  ModelName=talos_navigation  BlockId=ParamGet_talos_navigation_255
  diagnostics : Outport
  wires:
  heading_std_warning/1 -> diagnostics_bus/1  "heading_std_warning"
  position_offset_warning/1 -> diagnostics_bus/2  "position_offset_warning"
  diagnostics_period/1 -> diagnostics_bus/3  "diagnostics_period"
  publish_debug_diagnostics/1 -> diagnostics_bus/4  "publish_debug_diagnostics"
  diagnostics_bus/1 -> diagnostics/1
